simulink model "ControlE"  (R2024b)
settings: Solver=VariableStepAuto  StartTime=0.0  StopTime=115  RelTol=1e-3
InitFcn:
  | run("trajectory_q_8.m")
StopFcn:
  | run("vidControlE.m")
settings Model: Creator=mery  LastModifiedBy=genni

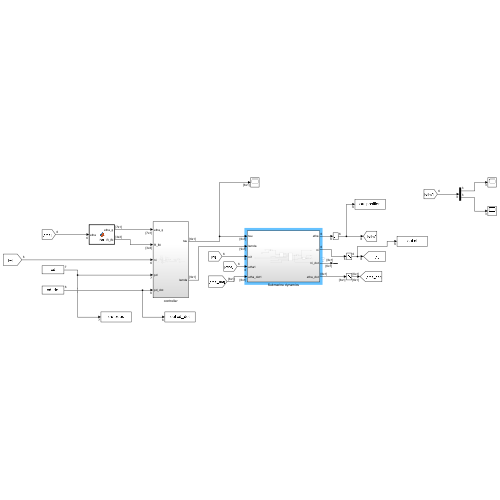
[thumbnail: Simulink's stored preview of the top-level diagram]
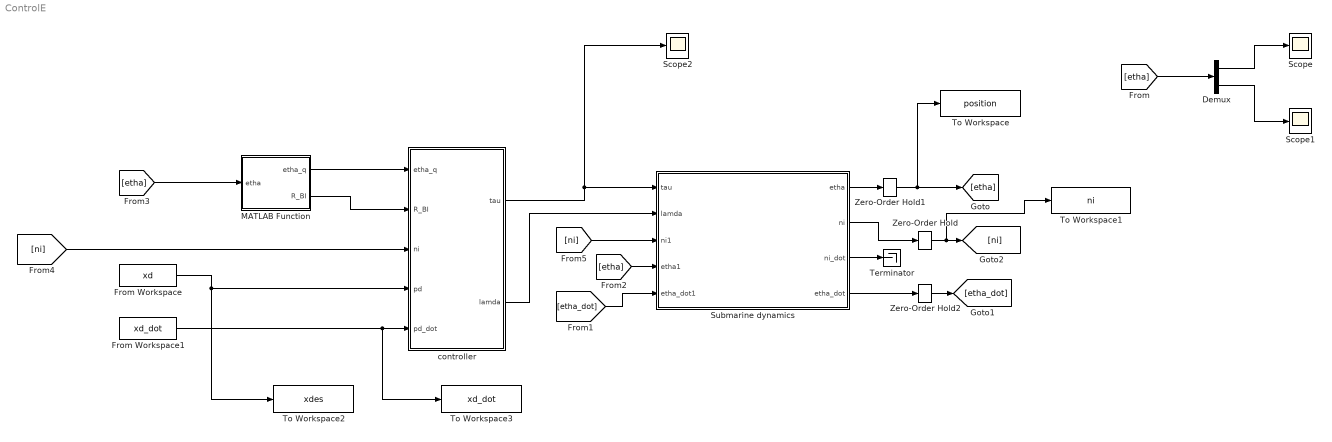
== system ControlE ==
  Demux : Demux  Outputs=2
  From Workspace : FromWorkspace  VariableName=xd  SampleTime=0.001
  From Workspace1 : FromWorkspace  VariableName=xd_dot  SampleTime=0.001
  MATLAB Function : MATLAB Function  TreatAsAtomicUnit=on
  Scope : Scope
  Scope1 : Scope
  Scope2 : Scope
  Submarine dynamics : Subsystem
  Terminator : Terminator
  To Workspace : ToWorkspace  VariableName=position  SaveFormat=Timeseries  SampleTime=-1
  To Workspace1 : ToWorkspace  VariableName=ni  SaveFormat=Timeseries  SampleTime=-1
  To Workspace2 : ToWorkspace  VariableName=xdes  SaveFormat=Timeseries  SampleTime=-1
  To Workspace3 : ToWorkspace  VariableName=xd_dot  SaveFormat=Timeseries  SampleTime=-1
  Zero-Order Hold : ZeroOrderHold  SampleTime=0.001
  Zero-Order Hold1 : ZeroOrderHold  SampleTime=0.001
  Zero-Order Hold2 : ZeroOrderHold  SampleTime=0.001
  controller : Subsystem
  wires:
  Submarine dynamics/2(ni) -> Zero-Order Hold/1
  Submarine dynamics/3(ni_dot) -> Terminator/1
  From Workspace/1 -> To Workspace2/1, controller/4(pd)
  From Workspace1/1 -> To Workspace3/1, controller/5(pd_dot)
  Demux/1 -> Scope/1
  Demux/2 -> Scope1/1
  controller/2(lamda) -> Submarine dynamics/2(lamda)
  Submarine dynamics/4(etha_dot) -> Zero-Order Hold2/1
  Submarine dynamics/1(etha) -> Zero-Order Hold1/1
  MATLAB Function/1(etha_q) -> controller/1(etha_q)
  MATLAB Function/2(R_BI) -> controller/2(R_BI)
  controller/1(tau) -> Scope2/1, Submarine dynamics/1(tau)
  Zero-Order Hold1/1 -> To Workspace/1, [etha]
  [etha] -> Demux/1
  [etha] -> MATLAB Function/1(etha)
  [etha] -> Submarine dynamics/4(etha1)
  Zero-Order Hold2/1 -> [etha_dot]
  [etha_dot] -> Submarine dynamics/5(etha_dot1)
  [ni] -> controller/3(ni)
  Zero-Order Hold/1 -> To Workspace1/1, [ni]
  [ni] -> Submarine dynamics/3(ni1)

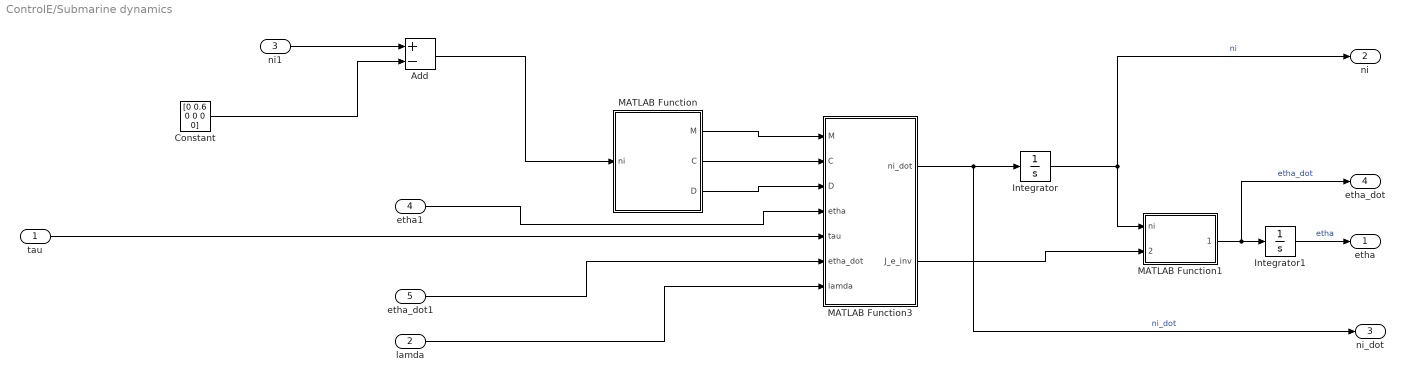
== system ControlE/Submarine dynamics ==
  tau : Inport
  lamda : Inport  Port=2
  ni1 : Inport  Port=3
  etha1 : Inport  Port=4
  etha_dot1 : Inport  Port=5
  Add : Sum  Inputs=+-
  Constant : Constant  Value=[0 0.6 0 0 0 0]
  Integrator : Integrator  InitialCondition=[0; 0; 0; 0; 0; 0]
  Integrator1 : Integrator  InitialCondition=[1; 0; 0; 0; 0; 0]
  MATLAB Function : MATLAB Function  TreatAsAtomicUnit=on
  MATLAB Function1 : MATLAB Function  TreatAsAtomicUnit=on
  MATLAB Function3 : MATLAB Function  TreatAsAtomicUnit=on
  etha : Outport
  ni : Outport  Port=2
  ni_dot : Outport  Port=3
  etha_dot : Outport  Port=4
  wires:
  Integrator/1 -> MATLAB Function1/1(ni), ni/1  "ni"
  MATLAB Function/1(M) -> MATLAB Function3/1(M)
  MATLAB Function/2(C) -> MATLAB Function3/2(C)
  MATLAB Function/3(D) -> MATLAB Function3/3(D)
  MATLAB Function3/1(ni_dot) -> ni_dot/1, Integrator/1  "ni_dot"
  tau/1 -> MATLAB Function3/5(tau)
  MATLAB Function3/2(J_e_inv) -> MATLAB Function1/2(J_e_inv)
  MATLAB Function1/1(etha_dot) -> etha_dot/1, Integrator1/1  "etha_dot"
  Integrator1/1 -> etha/1  "etha"
  lamda/1 -> MATLAB Function3/7(lamda)
  etha1/1 -> MATLAB Function3/4(etha)
  etha_dot1/1 -> MATLAB Function3/6(etha_dot)
  Add/1 -> MATLAB Function/1(ni)
  ni1/1 -> Add/1
  Constant/1 -> Add/2

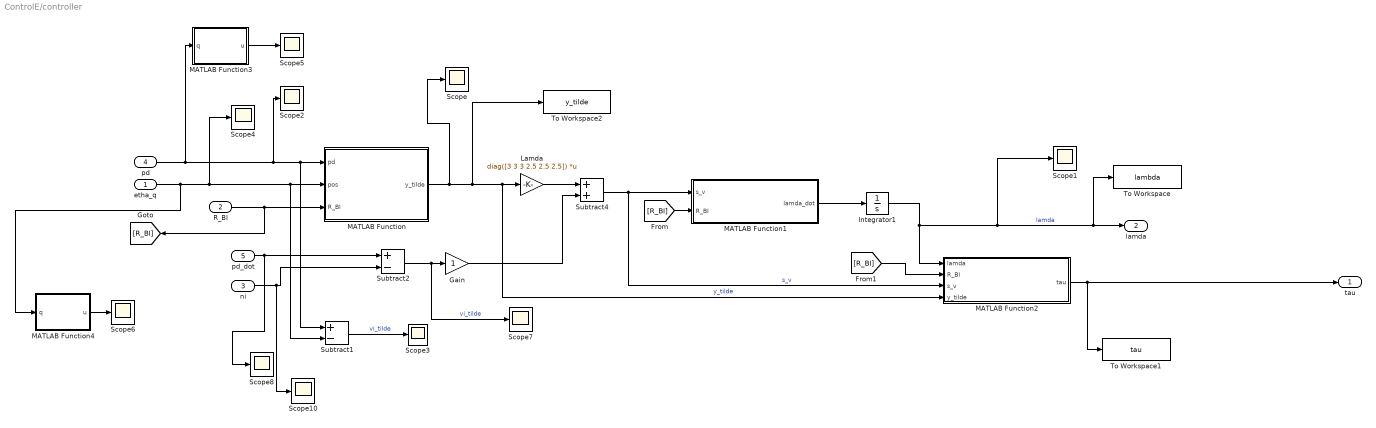
== system ControlE/controller ==
  etha_q : Inport
  R_BI : Inport  Port=2
  ni : Inport  Port=3
  pd : Inport  Port=4
  pd_dot : Inport  Port=5
  Gain : Gain
  Integrator1 : Integrator  InitialCondition=[0; 100; 0; 0; 0; 20; 0; 0; 0]
  Lamda : Gain  Gain=diag([3 3 3 2.5 2.5 2.5])  Multiplication=Matrix(K*u)
  MATLAB Function : MATLAB Function  TreatAsAtomicUnit=on
  MATLAB Function1 : MATLAB Function  TreatAsAtomicUnit=on
  MATLAB Function2 : MATLAB Function  TreatAsAtomicUnit=on
  MATLAB Function3 : MATLAB Function  TreatAsAtomicUnit=on
  MATLAB Function4 : MATLAB Function  TreatAsAtomicUnit=on
  Scope{,1..8,10} (10 alike) : Scope
  Subtract1 : Sum  Inputs=+-
  Subtract2 : Sum  Inputs=+-
  Subtract4 : Sum
  To Workspace : ToWorkspace  VariableName=lambda  SaveFormat=Timeseries  SampleTime=-1
  To Workspace1 : ToWorkspace  VariableName=tau  SaveFormat=Timeseries  SampleTime=-1
  To Workspace2 : ToWorkspace  VariableName=y_tilde  SaveFormat=Timeseries  SampleTime=-1
  tau : Outport
  lamda : Outport  Port=2
  wires:
  pd_dot/1 -> Scope8/1, Subtract2/1
  ni/1 -> Scope10/1, Subtract2/2
  pd/1 -> MATLAB Function3/1(q), Scope2/1, Subtract1/1, MATLAB Function/1(pd)
  Lamda/1 -> Subtract4/1
  Subtract4/1 -> MATLAB Function2/3(s_v), MATLAB Function1/1(s_v)  "s_v"
  MATLAB Function1/1(lamda_dot) -> Integrator1/1
  Integrator1/1 -> MATLAB Function2/1(lamda), Scope1/1, To Workspace/1, lamda/1  "lamda"
  MATLAB Function2/1(tau) -> To Workspace1/1, tau/1
  MATLAB Function/1(y_tilde) -> Scope/1, To Workspace2/1, MATLAB Function2/4(y_tilde), Lamda/1  "y_tilde"
  R_BI/1 -> MATLAB Function/3(R_BI), [R_BI]
  [R_BI] -> MATLAB Function1/2(R_BI)
  [R_BI] -> MATLAB Function2/2(R_BI)
  MATLAB Function3/1(u) -> Scope5/1
  Subtract2/1 -> Scope7/1, Gain/1  "vi_tilde"
  Gain/1 -> Subtract4/2
  Subtract1/1 -> Scope3/1  "vi_tilde"
  MATLAB Function4/1(u) -> Scope6/1
  etha_q/1 -> MATLAB Function4/1(q), Scope4/1, Subtract1/2, MATLAB Function/2(pos)

== matlab function ControlE/Submarine dynamics/MATLAB Function1 ==
  data: ni input; etha_dot output; J_e_inv input
function etha_dot = fcn(ni,J_e_inv)



etha_dot=J_e_inv*ni;

== matlab function ControlE/Submarine dynamics/MATLAB Function ==
  data: ni input; M output; C output; D output
function [M,C,D] = fcn(ni)

u1=ni(1:3);
u2=ni(4:6);
a=0.6;
b=0.3;
c=0.3;
e_c=0.75;
mass=225;
g=9.81;
r_g=[0 0 0]';
r_b=[0 0 0.05]';
W=mass*g;
B=2219;
I_0=[8 0 0
    0 20 0
    0 0 20];
M_rb=[mass*eye(3) -mass*skew(r_g)
    mass*skew(r_g) I_0];

X_u_dot=-67;
Y_v_dot=-140;
Z_w_dot=-140;
K_p_dot=0;
M_q_dot=-2.5;
N_r_dot=-2.5;

M_a=diag([-X_u_dot -Y_v_dot -Z_w_dot -K_p_dot -M_q_dot -N_r_dot]);

M=M_rb+M_a;

C_rb=[zeros(3) -mass*skew(u1)-mass*skew(skew(u2)*r_g);
    -mass*skew(u1)-mass*skew(skew(u2)*r_g) mass*skew(skew(u2)*r_g)-skew(I_0*u2)];

u=u1(1);
v=u1(2);
w=u1(3);

p=u2(1);
q=u2(2);
r=u2(3);

C_a=[0 0 0 0 -Z_w_dot*w Y_v_dot*v
    0 0 0 Z_w_dot*w 0 -X_u_dot*u
    0 0 0 -Y_v_dot*v X_u_dot*u 0
    0 -Z_w_dot*w Y_v_dot*v 0 -N_r_dot*r M_q_dot*q
    Z_w_dot*w 0 -X_u_dot*u N_r_dot*r 0 -K_p_dot*p
    -Y_v_dot*v X_u_dot*u 0 -M_q_dot*q K_p_dot*p 0];

C=C_rb+C_a;

X_u_u=50;
Y_v_v=-100;
Z_w_w=-100;
K_p_p=-10;
M_q_q=-80;
N_r_r=-80;
K_p=-5;
M_q=-20;
N_r=-20;

D=diag([X_u_u*abs(u) -Y_v_v*abs(v) -Z_w_w*abs(w) -K_p-K_p_p*abs(p) -M_q-M_q_q*abs(q) -N_r-N_r_r*abs(r)]);

== matlab function ControlE/controller/MATLAB Function ==
  data: pd input; y_tilde output; pos input; R_BI input
function y_tilde = fcn(pd,pos,R_BI)
etha1_des=pd(1:3);
etha2_des=pd(4:7);

etha1=pos(1:3);
etha2=pos(4:7);

etha1_tilde=etha1_des-etha1;

epsilon_tilde=pos(7)*pd(4:6)-pd(7)*pos(4:6)+skew(pos(4:6))*pd(4:6);

y_tilde=[R_BI*etha1_tilde
    epsilon_tilde];

== matlab function ControlE/Submarine dynamics/MATLAB Function3 ==
  data: M input; ni_dot output; C input; D input; etha input; tau input; etha_dot input; J_e_inv output; lamda input
function [ni_dot,J_e_inv] = fcn(M, C, D,etha,tau,etha_dot,lamda)

etha2=etha(4:6);

theta=etha2(2);
phi=etha2(1);
psi=etha2(3);

R_BI=[cos(psi)*cos(theta) sin(psi)*cos(theta) -sin(theta)
    -sin(psi)*cos(phi)+cos(psi)*sin(theta)*sin(phi) cos(psi)*cos(phi)+sin(psi)*sin(theta)*sin(phi) sin(phi)*cos(theta)
    sin(psi)*sin(phi)+cos(psi)*sin(theta)*cos(phi) -cos(psi)*sin(phi)+sin(psi)*sin(theta)*cos(phi) cos(phi)*cos(theta)];

J_k0=[1 0 -sin(theta)
    0 cos(phi) cos(theta)*sin(phi)
    0 -sin(phi) cos(theta)*cos(phi)];

J_e=[R_BI zeros(3,3)
    zeros(3,3) J_k0];

J_e_inv=inv(J_e);


ni=J_e*etha_dot;

g=9.81;
mass=225;
B=2219;
W=mass*g;

f_g=R_BI*[0;0;W];

f_b=-R_BI*[0;0;B];

r_g=[0 0 0]';
r_b=[0 0 0.05]';

g_RB=-[f_g+f_b
    cross(r_b,f_g)+cross(r_g,f_b)];


inversa=inv(M);

z=[0;0;1];

Phi=[zeros(3,3) R_BI zeros(3,3)
    skew(R_BI*z) zeros(3,3) R_BI];


% 
% ni_dot=inversa*(tau-C*ni-D*ni-Phi*lamda);
ni_dot=inversa*(tau-C*ni-D*ni-g_RB);

== matlab function ControlE/controller/MATLAB Function1 ==
  data: s_v input; lamda_dot output; R_BI input
function lamda_dot = fcn(s_v,R_BI)


z=[0;0;1];



Phi=[zeros(3,3) R_BI zeros(3,3)
    skew(R_BI*z) zeros(3,3) R_BI];

K_LP=16*eye(9);

lamda_dot=K_LP*Phi'*s_v;

== matlab function ControlE/controller/MATLAB Function2 ==
  data: lamda input; R_BI input; s_v input; y_tilde input; tau output
function tau= fcn(lamda,R_BI,s_v,y_tilde)



z=[0;0;1];



Phi=[zeros(3,3) R_BI zeros(3,3)
   skew(R_BI*z) zeros(3,3) R_BI];

K_D=diag([400 400 220  30 100 300]);

K=diag([100 100 100 0.1 100 100]);

tau=K_D*s_v+ K*y_tilde+ Phi*lamda;

== matlab function ControlE/MATLAB Function ==
  data: etha input; etha_q output; R_BI output
function [etha_q,R_BI] = fcn(etha)
etha2=etha(4:6);
etha1=etha(1:3);
theta=etha2(2);
phi=etha2(1);
psi=etha2(3);

R_BI=[cos(psi)*cos(theta) sin(psi)*cos(theta) -sin(theta)
    -sin(psi)*cos(phi)+cos(psi)*sin(theta)*sin(phi) cos(psi)*cos(phi)+sin(psi)*sin(theta)*sin(phi) sin(phi)*cos(theta)
    sin(psi)*sin(phi)+cos(psi)*sin(theta)*cos(phi) -cos(psi)*sin(phi)+sin(psi)*sin(theta)*cos(phi) cos(phi)*cos(theta)];


 etha_scalare=0.5*sqrt(R_BI(1,1)+R_BI(2,2)+R_BI(3,3)+1);
 
 epsilon_q=-0.5*[sign(R_BI(3,2)-R_BI(2,3))*sqrt(R_BI(1,1)-R_BI(2,2)-R_BI(3,3)+1)
        sign(R_BI(1,3)-R_BI(3,1))*sqrt(R_BI(2,2)-R_BI(3,3)-R_BI(1,1)+1)
        sign(R_BI(2,1)-R_BI(1,2))*sqrt(R_BI(3,3)-R_BI(2,2)-R_BI(1,1)+1)];

 etha_q=[etha1; epsilon_q; etha_scalare];

== matlab function ControlE/controller/MATLAB Function3 ==
  data: q input; u output
function u = fcn(q)

% Assicurati che q = [w, x, y, z]
    w = q(4); x = q(5); y = q(6); z = q(7);

    R = [1 - 2*(y^2 + x^2),     2*(x*w + z*y),       2*(w*y - x*z);
        2*(x*w - z*y),         1 - 2*(w^2 + y^2),   2*(y*x + z*w);
        2*(w*y + x*z),         2*(x*y - z*w),       1 - 2*(w^2 + x^2)];

    phi=atan2(R(3,2),R(3,3));

    theta=atan2(-R(3,1),sqrt(R(3,2)^2+R(3,3)^2));

    psi=atan2(R(2,1),R(1,1));

    u=[phi;theta;psi];

== matlab function ControlE/controller/MATLAB Function4 ==
  data: q input; u output
function u = fcn(q)

% Assicurati che q = [w, x, y, z]
    w = q(4); x = q(5); y = q(6); z = q(7);

    R = [1 - 2*(y^2 + x^2),     2*(x*w + z*y),       2*(w*y - x*z);
        2*(x*w - z*y),         1 - 2*(w^2 + y^2),   2*(y*x + z*w);
        2*(w*y + x*z),         2*(x*y - z*w),       1 - 2*(w^2 + x^2)];

    phi=atan2(R(3,2),R(3,3));

    theta=atan2(-R(3,1),sqrt(R(3,2)^2+R(3,3)^2));

    psi=atan2(R(2,1),R(1,1));

    u=[phi;theta;psi];
